simulink model "TB31_R2_ScPause_LoadStop"  (R2025a)
settings: Solver=FixedStepDiscrete  StartTime=0  StopTime=TB.t_end  FixedStep=TB.dt  RelTol=1e-3
InitFcn:
  | % 모델과 같은 폴더의 초기화 스크립트를 실행해 P(설계 파라미터)와 TB(시험 조건)를 만든다.
  | run(fullfile(fileparts(get_param(bdroot, 'FileName')), 'TB31_init.m'));
values from neighbouring files (symbols this model uses):
  TB = struct()    [TB31_init.m]    (also in run_TB31.m = evalin('base', 'TB'))
libraries: fl_lib x71, nesl_utility x31
(part 1 of 3)
settings Model: Creator=hj000  LastModifiedBy=hj000
settings DataIOCC: SaveOutput=off  SignalLogging=off  SaveTime=off

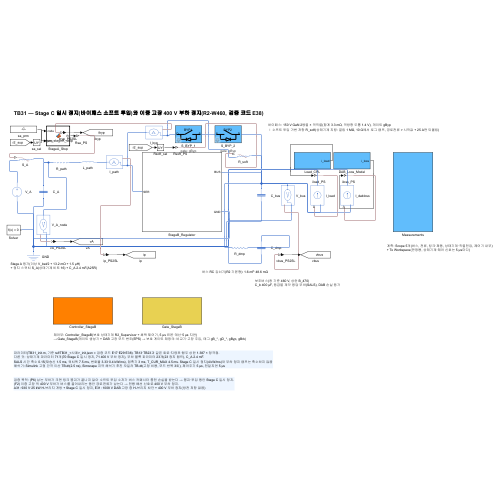
[thumbnail: Simulink's stored preview of the top-level diagram]
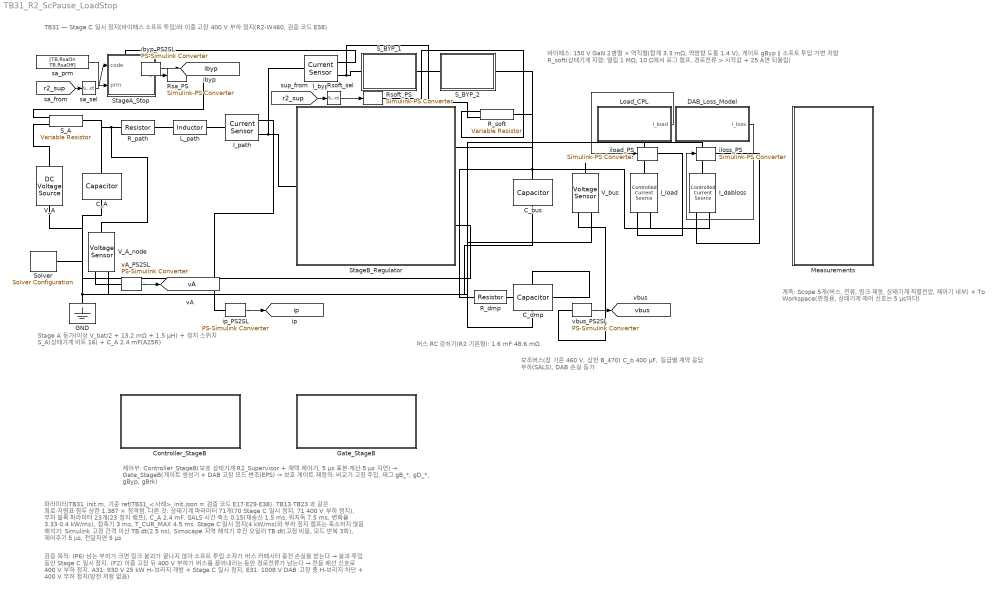
== system TB31_R2_ScPause_LoadStop ==
  note: TB31 — Stage C 일시 정지(바이패스 소프트 투입)와 이중 고장 400 V 부하 정지(R2-W460, 검증 코드 E38)
  note: Stage A 등가(이상 V_bat/2 + 13.2 mΩ + 1.5 µH)
      | + 정지 스위치 S_A(상태기계 비트 16) + C_A 2.4 mF(A25R)
  note: 바이패스: 150 V GaN 2병렬 × 역직렬(합계 3.3 mΩ, 역방향 도통 1.4 V), 게이트 gByp
      | ∥ 소프트 투입 가변 저항 R_soft(상태기계 지령: 열림 1 MΩ, 10 Ω에서 로그 램프, 경로전류 > 시작값 + 25 A면 되올림)
  note: 버스 RC 감쇠기(R2 기본형): 1.6 mF·48.6 mΩ
  note: 보조버스(창 기준 460 V, 상한 B_470)
      | C_b 400 µF, 등급별 계약 응답 부하(SALS), DAB 손실 등가
  note: 제어부: Controller_StageB(보호 상태기계 R2_Supervisor + 채택 제어기, 5 µs 표본·계산·5 µs 지연)
      | → Gate_StageB(게이트 생성기 + DAB 고장 모드 변조(EPS) → 보호 게이트 재정의: 비교기·고장 주입, 태그 gB_*, gD_*, gByp, gBrk)
  note: 계측: Scope 5개(버스, 전류, 링크·제동, 상태기계·직렬전압, 제어기 내부)
      | + To Workspace(판정용, 상태기계·제어 신호는 5 µs마다)
  note: 파라미터(TB31_init.m, 기준 ref/TB31_<사례>_init.json = 검증 코드 E17·E29·E38). TB13·TB23과 같은 회로·지령표·첨두 상한 1.387 × 정격점.
      | 다른 것: 상태기계 파라미터 71개(70 Stage C 일시 정지, 71 400 V 부하 정지), 부하 블록 파라미터 23개(23 정지 램프), C_A 2.4 mF.
      | SALS 시간 축소 0.15(재송신 1.5 ms, 워치독 7.5 ms, 변화율 3.33·0.4 kW/ms), 접촉기 3 ms, T_CUR_MAX 4.5 ms. Stage C 일시 정지(4 kW/ms)와 부하 정지 램프는 축소하지 않음
      | 해석기: Simulink 고정 간격 이산 TB.dt(2.5 ns), Simscape 지역 해석기 후진 오일러 TB.dt(고정 비용, 모드 반복 3회), 제어주기 5 µs, 전달지연 5 µs
  note: 검증 목적: (P6) 남는 부하가 크면 링크 붕괴가 끝나지 않아 소프트 투입 소자가 버스 커패시터 충전 손실을 받는다 → 붕괴·투입 동안 Stage C 일시 정지.
      | (F2) 이중 고장 뒤 400 V 부하가 버스를 끌어내리는 동안 경로전류가 남는다 → 전용 배선 신호로 400 V 부하 정지.
      | A31: 930 V·25 kW H-브리지 개방 + Stage C 일시 정지, E31: 1008 V DAB 고장 중 H-브리지 차단 + 400 V 부하 정지(방전 저항 없음)
  C_A : fl_lib/Electrical/Electrical Elements/Capacitor  c=TB.CA F  r=0 Ohm  g=0 1/Ohm  i_specify=off  i_priority=None  i=0 A  i_nominal_specify=off  i_nominal_value=1  i_nominal_unit=A  v_specify=off  v_priority=None  v=0 V  v_nominal_specify=off  v_nominal_value=1  v_nominal_unit=V  vc_specify=on  vc_priority=High  vc=TB.VA V  vc_nominal_specify=off  vc_nominal_value=1  vc_nominal_unit=V
  C_bus : fl_lib/Electrical/Electrical Elements/Capacitor  c=TB.Cb F  r=1e-6 Ohm  g=0 1/Ohm  i_specify=off  i_priority=None  i=0 A  i_nominal_specify=off  i_nominal_value=1  i_nominal_unit=A  v_specify=off  v_priority=None  v=0 V  v_nominal_specify=off  v_nominal_value=1  v_nominal_unit=V  vc_specify=on  vc_priority=High  vc=TB.vb0 V  vc_nominal_specify=off  vc_nominal_value=1  vc_nominal_unit=V
  C_dmp : fl_lib/Electrical/Electrical Elements/Capacitor  c=TB.Cdmp F  r=0 Ohm  g=0 1/Ohm  i_specify=off  i_priority=None  i=0 A  i_nominal_specify=off  i_nominal_value=1  i_nominal_unit=A  v_specify=off  v_priority=None  v=0 V  v_nominal_specify=off  v_nominal_value=1  v_nominal_unit=V  vc_specify=on  vc_priority=High  vc=TB.vcd0 V  vc_nominal_specify=off  vc_nominal_value=1  vc_nominal_unit=V
  Controller_StageB : Subsystem
  DAB_Loss_Model : Subsystem
  GND : fl_lib/Electrical/Electrical Elements/Electrical Reference
  Gate_StageB : Subsystem
  I_byp : fl_lib/Electrical/Electrical Sensors/Current Sensor
  I_dabloss : fl_lib/Electrical/Electrical Sources/Controlled Current Source
  I_load : fl_lib/Electrical/Electrical Sources/Controlled Current Source
  I_path : fl_lib/Electrical/Electrical Sensors/Current Sensor
  L_path : fl_lib/Electrical/Electrical Elements/Inductor  l=TB.Lpath H  r=0 Ohm  g=1e-9 1/Ohm  i_specify=off  i_priority=None  i=0 A  i_nominal_specify=off  i_nominal_value=1  i_nominal_unit=A  v_specify=off  v_priority=None  v=0 V  v_nominal_specify=off  v_nominal_value=1  v_nominal_unit=V  i_L_specify=on  i_L_priority=High  i_L=TB.ip0 A  i_L_nominal_specify=off  i_L_nominal_value=1  i_L_nominal_unit=A
  Load_CPL : Subsystem
  Measurements : Subsystem
  R_dmp : fl_lib/Electrical/Electrical Elements/Resistor  R=TB.Rdmp Ohm  i_specify=off  i_priority=None  i=0 A  i_nominal_specify=off  i_nominal_value=1  i_nominal_unit=A  v_specify=off  v_priority=None  v=0 V  v_nominal_specify=off  v_nominal_value=1  v_nominal_unit=V
  R_path : fl_lib/Electrical/Electrical Elements/Resistor  R=TB.Rpath Ohm  i_specify=off  i_priority=None  i=0 A  i_nominal_specify=off  i_nominal_value=1  i_nominal_unit=A  v_specify=off  v_priority=None  v=0 V  v_nominal_specify=off  v_nominal_value=1  v_nominal_unit=V
  R_soft : fl_lib/Electrical/Electrical Elements/Variable Resistor  Rmin=1e-4 Ohm  thermalEnable=false  thermal_mass=1 J/K  i_specify=off  i_priority=None  i=0 A  i_nominal_specify=off  i_nominal_value=1  i_nominal_unit=A  v_specify=off  v_priority=None  v=0 V  v_nominal_specify=off  v_nominal_value=1  v_nominal_unit=V  T_specify=off  T_priority=None  T=300 K  T_nominal_specify=off  T_nominal_value=1  T_nominal_unit=K
  Rsa_PS : nesl_utility/Simulink-PS Converter  PhysicalDomain=network_engine_domain  SubClassName=ps_input  LeftPortType=input  RightPortType=output  PseudoPeriodic=off  Frequencies=[]  NoiseDistribution=none  NoiseParameters=[]  Unit=1  AffineConversion=off  FilteringAndDerivatives=provide  SimscapeFilterOrder=1  InputFilterTimeConstant=0.001  UdotUserProvided=0
  Rsoft_PS : nesl_utility/Simulink-PS Converter  PhysicalDomain=network_engine_domain  SubClassName=ps_input  LeftPortType=input  RightPortType=output  PseudoPeriodic=off  Frequencies=[]  NoiseDistribution=none  NoiseParameters=[]  Unit=1  AffineConversion=off  FilteringAndDerivatives=provide  SimscapeFilterOrder=1  InputFilterTimeConstant=0.001  UdotUserProvided=0
  Rsoft_sel : Selector  InputPortWidth=12  IndexOptions=Index vector (dialog)  Indices=7  OutputSizes=1
  S_A : fl_lib/Electrical/Electrical Elements/Variable Resistor  Rmin=1e-5 Ohm  thermalEnable=false  thermal_mass=1 J/K  i_specify=off  i_priority=None  i=0 A  i_nominal_specify=off  i_nominal_value=1  i_nominal_unit=A  v_specify=off  v_priority=None  v=0 V  v_nominal_specify=off  v_nominal_value=1  v_nominal_unit=V  T_specify=off  T_priority=None  T=300 K  T_nominal_specify=off  T_nominal_value=1  T_nominal_unit=K
  S_BYP_1 : Subsystem  mask(PRISM-Hub switch cell){Ron=TB.Rbyp_cell, Goff=TB.B.Goff, Vf=TB.Vf_byp, Rd=TB.Rd_byp, Goffd=TB.B.Goffd}
      mask prompts: Ron "도통 저항 R_on [Ohm]"; Goff "차단 컨덕턴스 G_off [S]"; Vf "다이오드 순방향 전압 Vf [V]"; Rd "다이오드 도통 저항 R_d [Ohm]"; Goffd "다이오드 차단 컨덕턴스 [S]"
      mask help: 전력 반도체 스위치 셀 BYP1. 게이트 태그 gByp.
      settings: AttributesFormatString=gate: gByp
      mask Display:
      | plot([0.05 0.35 ],[0.50 0.50 ],[0.35 0.65 ],[0.50 0.74 ],[0.65 0.95 ],[0.50 0.50 ]);
      | plot([0.20 0.20 0.42 ],[0.50 0.20 0.20 ],[0.58 0.80 0.80 ],[0.20 0.20 0.50 ]);
      | plot([0.42 0.58 0.58 0.42 ],[0.20 0.10 0.30 0.20 ],[0.42 0.42 ],[0.10 0.30 ]);
      | text(0.5,0.80,'BYP1','horizontalAlignment','center','texmode','off');
      | port_label('LConn',1,'D');
      | port_label('RConn',1,'S');
  S_BYP_2 : Subsystem  mask(PRISM-Hub switch cell){Ron=TB.Rbyp_cell, Goff=TB.B.Goff, Vf=TB.Vf_byp, Rd=TB.Rd_byp, Goffd=TB.B.Goffd}
      mask prompts: Ron "도통 저항 R_on [Ohm]"; Goff "차단 컨덕턴스 G_off [S]"; Vf "다이오드 순방향 전압 Vf [V]"; Rd "다이오드 도통 저항 R_d [Ohm]"; Goffd "다이오드 차단 컨덕턴스 [S]"
      mask help: 전력 반도체 스위치 셀 BYP2. 게이트 태그 gByp.
      settings: AttributesFormatString=gate: gByp
      mask Display:
      | plot([0.95 0.65 ],[0.50 0.50 ],[0.65 0.35 ],[0.50 0.74 ],[0.35 0.05 ],[0.50 0.50 ]);
      | plot([0.80 0.80 0.58 ],[0.50 0.20 0.20 ],[0.42 0.20 0.20 ],[0.20 0.20 0.50 ]);
      | plot([0.58 0.42 0.42 0.58 ],[0.20 0.10 0.30 0.20 ],[0.58 0.58 ],[0.10 0.30 ]);
      | text(0.5,0.80,'BYP2','horizontalAlignment','center','texmode','off');
      | port_label('LConn',1,'D');
      | port_label('RConn',1,'S');
  Solver : nesl_utility/Solver Configuration  PhysicalDomain=network_engine_domain  SubClassName=solver  LeftPortType=input  RightPortType=generic  Tones=[]  Harmonics=[]  SimulateNoise=off  Profile=off  UseLocalSampling=off  EnableSwitchedLinearOptims=on  FrequencyDomain=off  UseCCode=off  RelTol=0.001  AbsTol=0.001  MinStep=1e-09  ToWorkspace=off  RevertToSquareIcSolve=off  NumHomotopyIterations=100  PhasorMode=off  PhasorModeNumHarmonics=1  ConsistencySolver=NEWTON_XTOL_AFTER_FTOL  IndexReductionMethod=DerivativeReplacement  DoDC=off  ResidualTolerance=1e-9  ConsistencyTolSource=GLOBAL  ConsistencyAbsTol=0.001  ConsistencyRelTol=0.001  ConsistencyTolFactor=0.001  UseLocalSolver=on  LocalSolverChoice=NE_BACKWARD_EULER_ADVANCER  ResolveIndetEquations=on  FunctionEvalNumThread=1  LocalSolverSampleTime=TB.dt  DoFixedCost=on  MaxNonlinIter=3  MaxModeIter=2  ComputeImpulses=off  ImpulseIterations=2  LinearAlgebra=auto  LinearAlgebraNumThread=0  EquationFormulation=NE_TIME_EF  DelaysMemoryBudget=1024  AutomaticFiltering=on  FilteringTimeConstant=0.001  PartitionStorageMethod=AS_NEEDED  PartitionMemoryBudget=1024  PartitionMethod=ROBUST  MultibodyUseLocalSolver=off  MultibodyLocalSolverChoice=ODE1  MultibodyLocalSolverSampleTime=0.001
  StageA_Stop : MATLAB Function  TreatAsAtomicUnit=on
  StageB_Regulator : Subsystem
  V_A : fl_lib/Electrical/Electrical Sources/DC Voltage Source  v0=TB.VA V
  V_A_node : fl_lib/Electrical/Electrical Sensors/Voltage Sensor
  V_bus : fl_lib/Electrical/Electrical Sensors/Voltage Sensor
  ibyp_PS2SL : nesl_utility/PS-Simulink Converter  PhysicalDomain=network_engine_domain  SubClassName=ps_output  LeftPortType=input  RightPortType=output  PseudoPeriodic=off  Frequencies=[]  VectorFormat=inherit  Unit=inherit  AffineConversion=off
  iload_PS : nesl_utility/Simulink-PS Converter  PhysicalDomain=network_engine_domain  SubClassName=ps_input  LeftPortType=input  RightPortType=output  PseudoPeriodic=off  Frequencies=[]  NoiseDistribution=none  NoiseParameters=[]  Unit=1  AffineConversion=off  FilteringAndDerivatives=provide  SimscapeFilterOrder=1  InputFilterTimeConstant=0.001  UdotUserProvided=0
  iloss_PS : nesl_utility/Simulink-PS Converter  PhysicalDomain=network_engine_domain  SubClassName=ps_input  LeftPortType=input  RightPortType=output  PseudoPeriodic=off  Frequencies=[]  NoiseDistribution=none  NoiseParameters=[]  Unit=1  AffineConversion=off  FilteringAndDerivatives=provide  SimscapeFilterOrder=1  InputFilterTimeConstant=0.001  UdotUserProvided=0
  ip_PS2SL : nesl_utility/PS-Simulink Converter  PhysicalDomain=network_engine_domain  SubClassName=ps_output  LeftPortType=input  RightPortType=output  PseudoPeriodic=off  Frequencies=[]  VectorFormat=inherit  Unit=inherit  AffineConversion=off
  sa_prm : Constant  Value=[TB.RsaOn TB.RsaOff]
  sa_sel : Selector  InputPortWidth=12  IndexOptions=Index vector (dialog)  Indices=10  OutputSizes=1
  vA_PS2SL : nesl_utility/PS-Simulink Converter  PhysicalDomain=network_engine_domain  SubClassName=ps_output  LeftPortType=input  RightPortType=output  PseudoPeriodic=off  Frequencies=[]  VectorFormat=inherit  Unit=inherit  AffineConversion=off
  vbus_PS2SL : nesl_utility/PS-Simulink Converter  PhysicalDomain=network_engine_domain  SubClassName=ps_output  LeftPortType=input  RightPortType=output  PseudoPeriodic=off  Frequencies=[]  VectorFormat=inherit  Unit=inherit  AffineConversion=off
  tag scope: ibyp=global, ip=global, vA=global, vbus=global
  wires:
  [r2_sup] -> sa_sel/1
  sa_sel/1 -> StageA_Stop/1(code)
  sa_prm/1 -> StageA_Stop/2(prm)
  StageA_Stop/1(R) -> Rsa_PS/1
  [r2_sup] -> Rsoft_sel/1
  Rsoft_sel/1 -> Rsoft_PS/1
  ip_PS2SL/1 -> [ip]
  vbus_PS2SL/1 -> [vbus]
  ibyp_PS2SL/1 -> [ibyp]
  vA_PS2SL/1 -> [vA]
  Load_CPL/1(i_load) -> iload_PS/1
  DAB_Loss_Model/1(i_loss) -> iloss_PS/1
  connections:
  Solver/RConn1 -- C_A/RConn1 -- V_A_node/RConn2 -- V_A/RConn1 -- StageB_Regulator/RConn2 -- C_bus/RConn1 -- C_dmp/RConn1 -- V_bus/RConn2 -- I_load/LConn1 -- GND/LConn1 -- I_dabloss/LConn1
  V_A/LConn1 -- S_A/LConn2
  S_A/RConn1 -- C_A/LConn1 -- R_path/LConn1 -- V_A_node/LConn1
  Rsa_PS/RConn1 -- S_A/LConn1
  R_path/RConn1 -- L_path/LConn1
  L_path/RConn1 -- I_path/LConn1
  StageB_Regulator/LConn1 -- I_path/RConn2 -- I_byp/LConn1
  S_BYP_1/LConn1 -- I_byp/RConn2 -- R_soft/LConn2
  S_BYP_1/RConn1 -- S_BYP_2/RConn1
  S_BYP_2/LConn1 -- R_soft/RConn1 -- StageB_Regulator/RConn1 -- R_dmp/LConn1 -- V_bus/LConn1 -- I_load/RConn2 -- C_bus/LConn1 -- I_dabloss/RConn2
  Rsoft_PS/RConn1 -- R_soft/LConn1
  R_dmp/RConn1 -- C_dmp/LConn1
  iload_PS/RConn1 -- I_load/RConn1
  iloss_PS/RConn1 -- I_dabloss/RConn1
  I_path/RConn1 -- ip_PS2SL/LConn1
  V_bus/RConn1 -- vbus_PS2SL/LConn1
  I_byp/RConn1 -- ibyp_PS2SL/LConn1
  V_A_node/RConn1 -- vA_PS2SL/LConn1

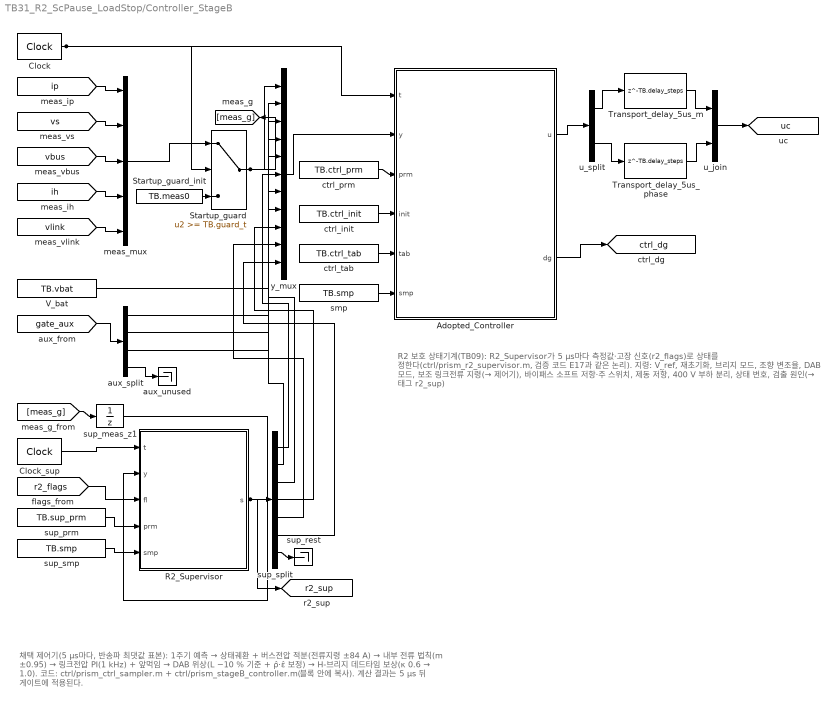
== system TB31_R2_ScPause_LoadStop/Controller_StageB ==
  note: R2 보호 상태기계(TB09): R2_Supervisor가 5 µs마다 측정값·고장 신호(r2_flags)로 상태를 정한다(ctrl/prism_r2_supervisor.m,
      | 검증 코드 E17과 같은 논리). 지령: V_ref, 재초기화, 브리지 모드, 조향 변조율, DAB 모드, 보조 링크전류 지령(→ 제어기),
      | 바이패스 소프트 저항·주 스위치, 제동 저항, 400 V 부하 분리, 상태 번호, 검출 원인(→ 태그 r2_sup)
  note: 채택 제어기(5 µs마다, 반송파 최댓값 표본): 1주기 예측 → 상태궤환 + 버스전압 적분(전류지령 ±84 A) → 내부 전류 법칙(m ±0.95)
      | → 링크전압 PI(1 kHz) + 앞먹임 → DAB 위상(L −10 % 기준 + ρ̂·ε̂ 보정) → H-브리지 데드타임 보상(κ 0.6 → 1.0).
      | 코드: ctrl/prism_ctrl_sampler.m + ctrl/prism_stageB_controller.m(블록 안에 복사). 계산 결과는 5 µs 뒤 게이트에 적용된다.
  Adopted_Controller : MATLAB Function  TreatAsAtomicUnit=on
  Clock : DigitalClock  SampleTime=TB.dt
  Clock_sup : DigitalClock  SampleTime=TB.dt
  R2_Supervisor : MATLAB Function  TreatAsAtomicUnit=on
  Startup_guard : Switch  Threshold=TB.guard_t  SaturateOnIntegerOverflow=off  InputSameDT=off
  Startup_guard_init : Constant  Value=TB.meas0
  Transport_delay_5us_m : Delay  DelayLength=TB.delay_steps  InitialCondition=TB.uc0(1)
  Transport_delay_5us_phase : Delay  DelayLength=TB.delay_steps  InitialCondition=TB.uc0(2)
  V_bat : Constant  Value=TB.vbat
  aux_split : Demux  Outputs=[1 1 1 3]
  aux_unused : Terminator
  ctrl_init : Constant  Value=TB.ctrl_init
  ctrl_prm : Constant  Value=TB.ctrl_prm
  ctrl_tab : Constant  Value=TB.ctrl_tab
  meas_mux : Mux  Inputs=5
  smp : Constant  Value=TB.smp
  sup_meas_z1 : UnitDelay  InitialCondition=TB.meas0'  SampleTime=TB.dt  HasFrameUpgradeWarning=on
  sup_prm : Constant  Value=TB.sup_prm
  sup_rest : Terminator
  sup_smp : Constant  Value=TB.smp
  sup_split : Demux  Outputs=[1 1 1 1 1 1 6]
  u_join : Mux  Inputs=2
  u_split : Demux  Outputs=2
  y_mux : Mux  Inputs=11
  tag scope: ctrl_dg=global, r2_sup=global, uc=global
  wires:
  [ip] -> meas_mux/1
  [vs] -> meas_mux/2
  [vbus] -> meas_mux/3
  [ih] -> meas_mux/4
  [vlink] -> meas_mux/5
  Startup_guard_init/1 -> Startup_guard/3
  meas_mux/1 -> Startup_guard/1
  Clock/1 -> Startup_guard/2, Adopted_Controller/1(t)
  Startup_guard/1 -> y_mux/1, [meas_g]
  V_bat/1 -> y_mux/2
  [gate_aux] -> aux_split/1
  aux_split/1 -> y_mux/3
  aux_split/2 -> y_mux/4
  aux_split/3 -> y_mux/5
  aux_split/4 -> aux_unused/1
  Clock_sup/1 -> R2_Supervisor/1(t)
  [meas_g] -> sup_meas_z1/1
  sup_meas_z1/1 -> R2_Supervisor/2(y)
  [r2_flags] -> R2_Supervisor/3(fl)
  sup_prm/1 -> R2_Supervisor/4(prm)
  sup_smp/1 -> R2_Supervisor/5(smp)
  R2_Supervisor/1(s) -> [r2_sup], sup_split/1
  sup_split/1 -> y_mux/6
  sup_split/2 -> y_mux/7
  sup_split/3 -> y_mux/8
  sup_split/4 -> y_mux/9
  sup_split/5 -> y_mux/10
  sup_split/6 -> y_mux/11
  sup_split/7 -> sup_rest/1
  y_mux/1 -> Adopted_Controller/2(y)
  ctrl_prm/1 -> Adopted_Controller/3(prm)
  ctrl_init/1 -> Adopted_Controller/4(init)
  ctrl_tab/1 -> Adopted_Controller/5(tab)
  smp/1 -> Adopted_Controller/6(smp)
  Adopted_Controller/1(u) -> u_split/1
  u_split/1 -> Transport_delay_5us_m/1
  u_split/2 -> Transport_delay_5us_phase/1
  Transport_delay_5us_m/1 -> u_join/1
  Transport_delay_5us_phase/1 -> u_join/2
  u_join/1 -> [uc]
  Adopted_Controller/2(dg) -> [ctrl_dg]

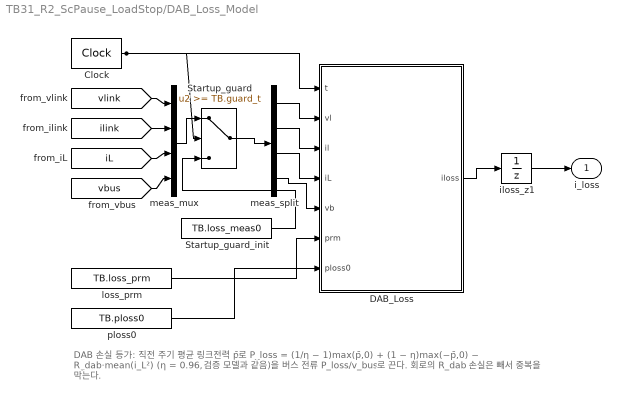
== system TB31_R2_ScPause_LoadStop/DAB_Loss_Model ==
  note: DAB 손실 등가: 직전 주기 평균 링크전력 p̄로 P_loss = (1/η − 1)max(p̄,0) + (1 − η)max(−p̄,0) − R_dab·mean(i_L²)
      | (η = 0.96, 검증 모델과 같음)을 버스 전류 P_loss/v_bus로 끈다. 회로의 R_dab 손실은 빼서 중복을 막는다.
  Clock : DigitalClock  SampleTime=TB.dt
  DAB_Loss : MATLAB Function  TreatAsAtomicUnit=on
  Startup_guard : Switch  Threshold=TB.guard_t  SaturateOnIntegerOverflow=off  InputSameDT=off
  Startup_guard_init : Constant  Value=TB.loss_meas0
  iloss_z1 : UnitDelay  SampleTime=TB.dt  HasFrameUpgradeWarning=on
  loss_prm : Constant  Value=TB.loss_prm
  meas_mux : Mux
  meas_split : Demux
  ploss0 : Constant  Value=TB.ploss0
  i_loss : Outport
  wires:
  [vlink] -> meas_mux/1
  [ilink] -> meas_mux/2
  [iL] -> meas_mux/3
  [vbus] -> meas_mux/4
  Startup_guard_init/1 -> Startup_guard/3
  meas_mux/1 -> Startup_guard/1
  Clock/1 -> Startup_guard/2, DAB_Loss/1(t)
  Startup_guard/1 -> meas_split/1
  meas_split/1 -> DAB_Loss/2(vl)
  meas_split/2 -> DAB_Loss/3(il)
  meas_split/3 -> DAB_Loss/4(iL)
  meas_split/4 -> DAB_Loss/5(vb)
  loss_prm/1 -> DAB_Loss/6(prm)
  ploss0/1 -> DAB_Loss/7(ploss0)
  DAB_Loss/1(iloss) -> iloss_z1/1
  iloss_z1/1 -> i_loss/1

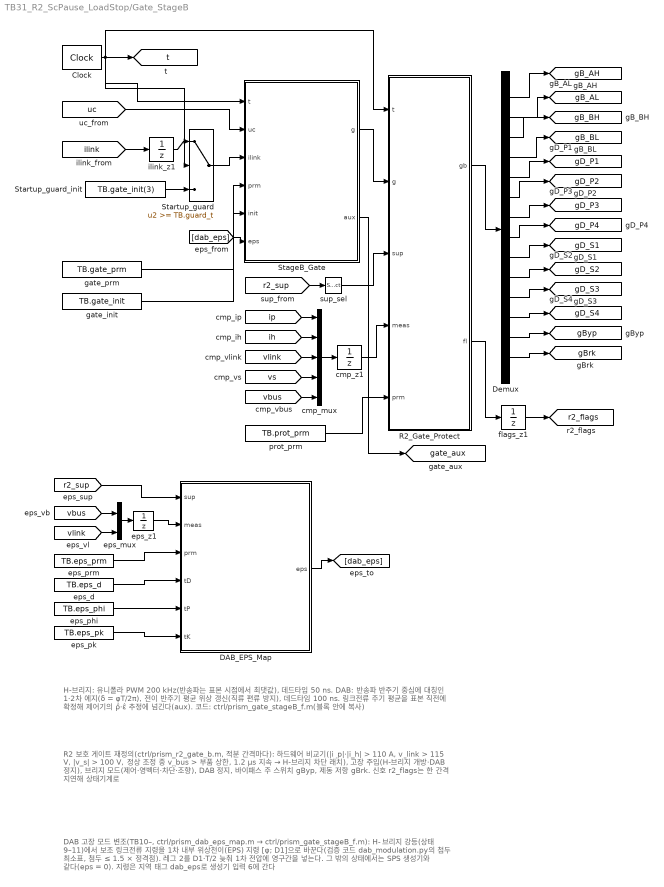
== system TB31_R2_ScPause_LoadStop/Gate_StageB ==
  note: H-브리지: 유니폴라 PWM 200 kHz(반송파는 표본 시점에서 최댓값), 데드타임 50 ns.
      | DAB: 반송파 반주기 중심에 대칭인 1·2차 에지(δ = φT/2π), 전이 반주기 평균 위상 갱신(직류 편류 방지), 데드타임 100 ns.
      | 링크전류 주기 평균을 표본 직전에 확정해 제어기의 ρ̂·ε̂ 추정에 넘긴다(aux). 코드: ctrl/prism_gate_stageB_f.m(블록 안에 복사)
  note: DAB 고장 모드 변조(TB10–, ctrl/prism_dab_eps_map.m → ctrl/prism_gate_stageB_f.m): H-브리지 강등(상태 9–11)에서 보조 링크전류 지령을
      | 1차 내부 위상천이(EPS) 지령 [φ; D1]으로 바꾼다(검증 코드 dab_modulation.py의 첨두 최소표, 첨두 ≤ 1.5 × 정격점). 레그 2를 D1·T/2 늦춰
      | 1차 전압에 영구간을 넣는다. 그 밖의 상태에서는 SPS 생성기와 같다(eps = 0). 지령은 지역 태그 dab_eps로 생성기 입력 6에 간다
  note: R2 보호 게이트 재정의(ctrl/prism_r2_gate_b.m, 적분 간격마다): 하드웨어 비교기(|i_p|·|i_h| > 110 A, v_link > 115 V,
      | |v_s| > 100 V, 정상 조정 중 v_bus > 부품 상한, 1.2 µs 지속 → H-브리지 차단 래치), 고장 주입(H-브리지 개방·DAB 정지),
      | 브리지 모드(제어·영벡터·차단·조향), DAB 정지, 바이패스 주 스위치 gByp, 제동 저항 gBrk. 신호 r2_flags는 한 간격 지연해 상태기계로
  Clock : DigitalClock  SampleTime=TB.dt
  DAB_EPS_Map : MATLAB Function  TreatAsAtomicUnit=on
  Demux : Demux  Outputs=14
  R2_Gate_Protect : MATLAB Function  TreatAsAtomicUnit=on
  StageB_Gate : MATLAB Function  TreatAsAtomicUnit=on
  Startup_guard : Switch  Threshold=TB.guard_t  SaturateOnIntegerOverflow=off  InputSameDT=off
  Startup_guard_init : Constant  Value=TB.gate_init(3)
  cmp_mux : Mux  Inputs=5
  cmp_z1 : UnitDelay  InitialCondition=[TB.ip0 TB.ih0 TB.vl0 TB.vs0 TB.vb0]'  SampleTime=TB.dt  HasFrameUpgradeWarning=on
  eps_d : Constant  Value=TB.eps_d
  eps_mux : Mux  Inputs=2
  eps_phi : Constant  Value=TB.eps_phi
  eps_pk : Constant  Value=TB.eps_pk
  eps_prm : Constant  Value=TB.eps_prm
  eps_z1 : UnitDelay  InitialCondition=[TB.vb0 TB.vl0]'  SampleTime=TB.dt  HasFrameUpgradeWarning=on
  flags_z1 : UnitDelay  SampleTime=TB.dt  HasFrameUpgradeWarning=on
  gate_init : Constant  Value=TB.gate_init
  gate_prm : Constant  Value=TB.gate_prm
  ilink_z1 : UnitDelay  SampleTime=TB.dt  HasFrameUpgradeWarning=on
  prot_prm : Constant  Value=TB.prot_prm
  sup_sel : Selector  InputPortWidth=12  IndexOptions=Index vector (dialog)  Indices=[3 5 8 9 11]  OutputSizes=1
  tag scope: gB_AH=global, gB_AL=global, gB_BH=global, gB_BL=global, gBrk=global, gByp=global, gD_P1=global, gD_P2=global, gD_P3=global, gD_P4=global, gD_S1=global, gD_S2=global, gD_S3=global, gD_S4=global, gate_aux=global, r2_flags=global, t=global
  wires:
  Startup_guard_init/1 -> Startup_guard/3
  Clock/1 -> [t], StageB_Gate/1(t), Startup_guard/2, R2_Gate_Protect/1(t)
  [uc] -> StageB_Gate/2(uc)
  [ilink] -> ilink_z1/1
  ilink_z1/1 -> Startup_guard/1
  Startup_guard/1 -> StageB_Gate/3(ilink)
  gate_prm/1 -> StageB_Gate/4(prm)
  gate_init/1 -> StageB_Gate/5(init)
  [r2_sup] -> sup_sel/1
  [ip] -> cmp_mux/1
  [ih] -> cmp_mux/2
  [vlink] -> cmp_mux/3
  [vs] -> cmp_mux/4
  [vbus] -> cmp_mux/5
  cmp_mux/1 -> cmp_z1/1
  StageB_Gate/1(g) -> R2_Gate_Protect/2(g)
  sup_sel/1 -> R2_Gate_Protect/3(sup)
  cmp_z1/1 -> R2_Gate_Protect/4(meas)
  prot_prm/1 -> R2_Gate_Protect/5(prm)
  R2_Gate_Protect/1(gb) -> Demux/1
  R2_Gate_Protect/2(fl) -> flags_z1/1
  flags_z1/1 -> [r2_flags]
  [vbus] -> eps_mux/1
  [vlink] -> eps_mux/2
  eps_mux/1 -> eps_z1/1
  [r2_sup] -> DAB_EPS_Map/1(sup)
  eps_z1/1 -> DAB_EPS_Map/2(meas)
  eps_prm/1 -> DAB_EPS_Map/3(prm)
  eps_d/1 -> DAB_EPS_Map/4(tD)
  eps_phi/1 -> DAB_EPS_Map/5(tP)
  eps_pk/1 -> DAB_EPS_Map/6(tK)
  DAB_EPS_Map/1(eps) -> [dab_eps]
  [dab_eps] -> StageB_Gate/6(eps)
  Demux/1 -> [gB_AH]
  Demux/2 -> [gB_AL]
  Demux/3 -> [gB_BH]
  Demux/4 -> [gB_BL]
  Demux/5 -> [gD_P1]
  Demux/6 -> [gD_P2]
  Demux/7 -> [gD_P3]
  Demux/8 -> [gD_P4]
  Demux/9 -> [gD_S1]
  Demux/10 -> [gD_S2]
  Demux/11 -> [gD_S3]
  Demux/12 -> [gD_S4]
  Demux/13 -> [gByp]
  Demux/14 -> [gBrk]
  StageB_Gate/2(aux) -> [gate_aux]

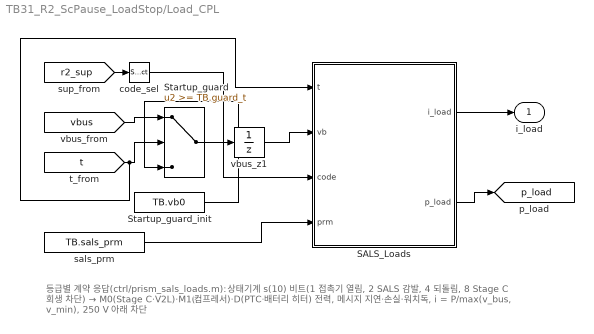
== system TB31_R2_ScPause_LoadStop/Load_CPL ==
  note: 등급별 계약 응답(ctrl/prism_sals_loads.m): 상태기계 s(10) 비트(1 접촉기 열림, 2 SALS 감발, 4 되돌림, 8 Stage C 회생 차단)
      | → M0(Stage C·V2L)·M1(컴프레서)·D(PTC·배터리 히터) 전력, 메시지 지연·손실·워치독, i = P/max(v_bus, v_min), 250 V 아래 차단
  SALS_Loads : MATLAB Function  TreatAsAtomicUnit=on
  Startup_guard : Switch  Threshold=TB.guard_t  SaturateOnIntegerOverflow=off  InputSameDT=off
  Startup_guard_init : Constant  Value=TB.vb0
  code_sel : Selector  InputPortWidth=12  IndexOptions=Index vector (dialog)  Indices=10  OutputSizes=1
  sals_prm : Constant  Value=TB.sals_prm
  vbus_z1 : UnitDelay  SampleTime=TB.dt  HasFrameUpgradeWarning=on
  i_load : Outport
  tag scope: p_load=global
  wires:
  [r2_sup] -> code_sel/1
  Startup_guard_init/1 -> Startup_guard/3
  [vbus] -> Startup_guard/1
  [t] -> Startup_guard/2, SALS_Loads/1(t)
  Startup_guard/1 -> vbus_z1/1
  vbus_z1/1 -> SALS_Loads/2(vb)
  code_sel/1 -> SALS_Loads/3(code)
  sals_prm/1 -> SALS_Loads/4(prm)
  SALS_Loads/1(i_load) -> i_load/1
  SALS_Loads/2(p_load) -> [p_load]

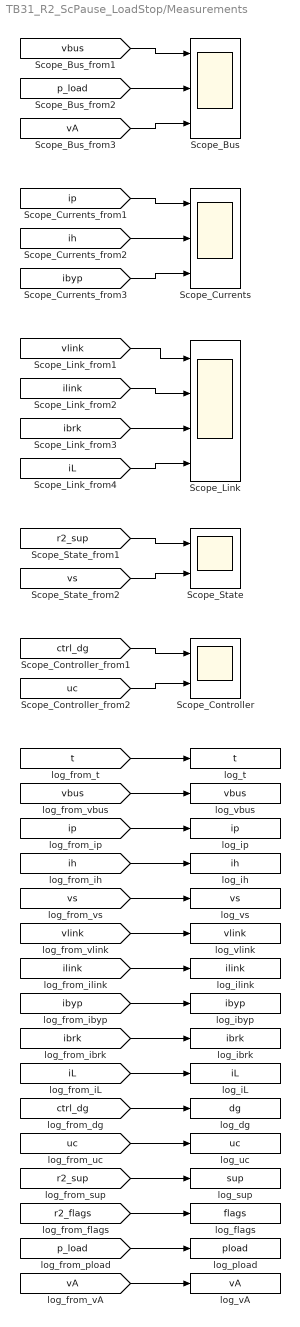
== system TB31_R2_ScPause_LoadStop/Measurements ==
  Scope_Bus : Scope  NumInputPorts=3
      settings: Title=Scope Bus
  Scope_Controller : Scope  NumInputPorts=2
      settings: Title=Scope Controller
  Scope_Currents : Scope  NumInputPorts=3
      settings: Title=Scope Currents
  Scope_Link : Scope  NumInputPorts=4
      settings: Title=Scope Link
  Scope_State : Scope  NumInputPorts=2
      settings: Title=Scope State
  log_dg : ToWorkspace  VariableName=dg  SampleTime=-1
      settings: Decimation=TB.Np
  log_flags : ToWorkspace  VariableName=flags  SampleTime=-1
      settings: Decimation=TB.Np
  log_iL : ToWorkspace  VariableName=iL  SampleTime=-1
  log_ibrk : ToWorkspace  VariableName=ibrk  SampleTime=-1
  log_ibyp : ToWorkspace  VariableName=ibyp  SampleTime=-1
  log_ih : ToWorkspace  VariableName=ih  SampleTime=-1
  log_ilink : ToWorkspace  VariableName=ilink  SampleTime=-1
  log_ip : ToWorkspace  VariableName=ip  SampleTime=-1
  log_pload : ToWorkspace  VariableName=pload  SampleTime=-1
      settings: Decimation=TB.Np
  log_sup : ToWorkspace  VariableName=sup  SampleTime=-1
      settings: Decimation=TB.Np
  log_t : ToWorkspace  VariableName=t  SampleTime=-1
  log_uc : ToWorkspace  VariableName=uc  SampleTime=-1
      settings: Decimation=TB.Np
  log_vA : ToWorkspace  VariableName=vA  SampleTime=-1
      settings: Decimation=TB.Np
  log_vbus : ToWorkspace  VariableName=vbus  SampleTime=-1
  log_vlink : ToWorkspace  VariableName=vlink  SampleTime=-1
  log_vs : ToWorkspace  VariableName=vs  SampleTime=-1
  wires:
  [vbus] -> Scope_Bus/1
  [p_load] -> Scope_Bus/2
  [vA] -> Scope_Bus/3
  [ip] -> Scope_Currents/1
  [ih] -> Scope_Currents/2
  [ibyp] -> Scope_Currents/3
  [vlink] -> Scope_Link/1
  [ilink] -> Scope_Link/2
  [ibrk] -> Scope_Link/3
  [iL] -> Scope_Link/4
  [r2_sup] -> Scope_State/1
  [vs] -> Scope_State/2
  [ctrl_dg] -> Scope_Controller/1
  [uc] -> Scope_Controller/2
  [t] -> log_t/1
  [vbus] -> log_vbus/1
  [ip] -> log_ip/1
  [ih] -> log_ih/1
  [vs] -> log_vs/1
  [vlink] -> log_vlink/1
  [ilink] -> log_ilink/1
  [ibyp] -> log_ibyp/1
  [ibrk] -> log_ibrk/1
  [iL] -> log_iL/1
  [ctrl_dg] -> log_dg/1
  [uc] -> log_uc/1
  [r2_sup] -> log_sup/1
  [r2_flags] -> log_flags/1
  [p_load] -> log_pload/1
  [vA] -> log_vA/1

== system TB31_R2_ScPause_LoadStop/S_BYP_1 ==
  note: 스위치 셀: 이상 스위치(R_on, G_off) + 역병렬 바디 다이오드(Vf, R_d)
      | 게이트: 전역 태그 "gByp" (> 0.5 이면 도통)
  D_body : fl_lib/Electrical/Electrical Elements/Diode  Vf=Vf V  Ron=Rd Ohm  Goff=Goffd 1/Ohm  i_specify=off  i_priority=None  i=0 A  i_nominal_specify=off  i_nominal_value=1  i_nominal_unit=A  v_specify=off  v_priority=None  v=0 V  v_nominal_specify=off  v_nominal_value=1  v_nominal_unit=V
  Gate_PS : nesl_utility/Simulink-PS Converter  PhysicalDomain=network_engine_domain  SubClassName=ps_input  LeftPortType=input  RightPortType=output  PseudoPeriodic=off  Frequencies=[]  NoiseDistribution=none  NoiseParameters=[]  Unit=1  AffineConversion=off  FilteringAndDerivatives=zero  SimscapeFilterOrder=1  InputFilterTimeConstant=0.001  UdotUserProvided=0
  SW : fl_lib/Electrical/Electrical Elements/Switch  R_closed=Ron Ohm  G_open=Goff 1/Ohm  Threshold=0.5  i_specify=off  i_priority=None  i=0 A  i_nominal_specify=off  i_nominal_value=1  i_nominal_unit=A  v_specify=off  v_priority=None  v=0 V  v_nominal_specify=off  v_nominal_value=1  v_nominal_unit=V
  D : PMIOPort  Side=Left
  S : PMIOPort  Port=2  Side=Right
  wires:
  [gByp] -> Gate_PS/1
  connections:
  Gate_PS/RConn1 -- SW/RConn1
  SW/LConn1 -- D/RConn1 -- D_body/RConn1
  S/RConn1 -- SW/RConn2 -- D_body/LConn1

== system TB31_R2_ScPause_LoadStop/S_BYP_2 ==
  note: 스위치 셀: 이상 스위치(R_on, G_off) + 역병렬 바디 다이오드(Vf, R_d)
      | 게이트: 전역 태그 "gByp" (> 0.5 이면 도통)
  D_body : fl_lib/Electrical/Electrical Elements/Diode  Vf=Vf V  Ron=Rd Ohm  Goff=Goffd 1/Ohm  i_specify=off  i_priority=None  i=0 A  i_nominal_specify=off  i_nominal_value=1  i_nominal_unit=A  v_specify=off  v_priority=None  v=0 V  v_nominal_specify=off  v_nominal_value=1  v_nominal_unit=V
  Gate_PS : nesl_utility/Simulink-PS Converter  PhysicalDomain=network_engine_domain  SubClassName=ps_input  LeftPortType=input  RightPortType=output  PseudoPeriodic=off  Frequencies=[]  NoiseDistribution=none  NoiseParameters=[]  Unit=1  AffineConversion=off  FilteringAndDerivatives=zero  SimscapeFilterOrder=1  InputFilterTimeConstant=0.001  UdotUserProvided=0
  SW : fl_lib/Electrical/Electrical Elements/Switch  R_closed=Ron Ohm  G_open=Goff 1/Ohm  Threshold=0.5  i_specify=off  i_priority=None  i=0 A  i_nominal_specify=off  i_nominal_value=1  i_nominal_unit=A  v_specify=off  v_priority=None  v=0 V  v_nominal_specify=off  v_nominal_value=1  v_nominal_unit=V
  D : PMIOPort  Side=Left
  S : PMIOPort  Port=2  Side=Right
  wires:
  [gByp] -> Gate_PS/1
  connections:
  Gate_PS/RConn1 -- SW/RConn1
  SW/LConn1 -- D/RConn1 -- D_body/RConn1
  S/RConn1 -- SW/RConn2 -- D_body/LConn1

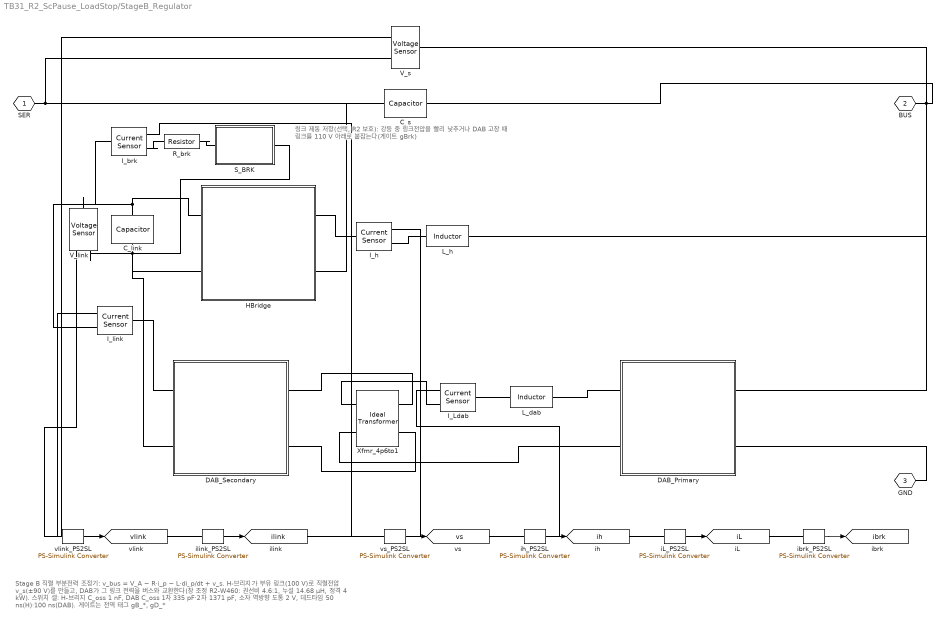
== system TB31_R2_ScPause_LoadStop/StageB_Regulator ==
  note: 링크 제동 저항(선택, R2 보호): 강등 중 링크전압을 빨리 낮추거나
      | DAB 고장 때 링크를 110 V 아래로 붙잡는다(게이트 gBrk)
  note: Stage B 직렬 부분전력 조정기: v_bus = V_A − R·i_p − L·di_p/dt + v_s.
      | H-브리지가 부유 링크(100 V)로 직렬전압 v_s(±90 V)를 만들고, DAB가 그 링크 전력을 버스와 교환한다(창 조정 R2-W460: 권선비 4.6:1, 누설 14.68 µH, 정격 4 kW).
      | 스위치 셀: H-브리지 C_oss 1 nF, DAB C_oss 1차 335 pF·2차 1371 pF, 소자 역방향 도통 2 V, 데드타임 50 ns(H)·100 ns(DAB). 게이트는 전역 태그 gB_*, gD_*
  C_link : fl_lib/Electrical/Electrical Elements/Capacitor  c=TB.B.Clink F  r=1e-6 Ohm  g=0 1/Ohm  i_specify=off  i_priority=None  i=0 A  i_nominal_specify=off  i_nominal_value=1  i_nominal_unit=A  v_specify=off  v_priority=None  v=0 V  v_nominal_specify=off  v_nominal_value=1  v_nominal_unit=V  vc_specify=on  vc_priority=High  vc=TB.vl0 V  vc_nominal_specify=off  vc_nominal_value=1  vc_nominal_unit=V
  C_s : fl_lib/Electrical/Electrical Elements/Capacitor  c=TB.B.Cs F  r=1e-6 Ohm  g=0 1/Ohm  i_specify=off  i_priority=None  i=0 A  i_nominal_specify=off  i_nominal_value=1  i_nominal_unit=A  v_specify=off  v_priority=None  v=0 V  v_nominal_specify=off  v_nominal_value=1  v_nominal_unit=V  vc_specify=on  vc_priority=High  vc=TB.vs0 V  vc_nominal_specify=off  vc_nominal_value=1  vc_nominal_unit=V
  DAB_Primary : Subsystem
  DAB_Secondary : Subsystem
  HBridge : Subsystem
  I_Ldab : fl_lib/Electrical/Electrical Sensors/Current Sensor
  I_brk : fl_lib/Electrical/Electrical Sensors/Current Sensor
  I_h : fl_lib/Electrical/Electrical Sensors/Current Sensor
  I_link : fl_lib/Electrical/Electrical Sensors/Current Sensor
  L_dab : fl_lib/Electrical/Electrical Elements/Inductor  l=TB.B.Ldab H  r=TB.B.Rdab Ohm  g=1e-9 1/Ohm  i_specify=off  i_priority=None  i=0 A  i_nominal_specify=off  i_nominal_value=1  i_nominal_unit=A  v_specify=off  v_priority=None  v=0 V  v_nominal_specify=off  v_nominal_value=1  v_nominal_unit=V  i_L_specify=on  i_L_priority=High  i_L=0 A  i_L_nominal_specify=off  i_L_nominal_value=1  i_L_nominal_unit=A
  L_h : fl_lib/Electrical/Electrical Elements/Inductor  l=TB.B.Lh H  r=TB.B.Rh Ohm  g=1e-9 1/Ohm  i_specify=off  i_priority=None  i=0 A  i_nominal_specify=off  i_nominal_value=1  i_nominal_unit=A  v_specify=off  v_priority=None  v=0 V  v_nominal_specify=off  v_nominal_value=1  v_nominal_unit=V  i_L_specify=on  i_L_priority=High  i_L=TB.ih0 A  i_L_nominal_specify=off  i_L_nominal_value=1  i_L_nominal_unit=A
  R_brk : fl_lib/Electrical/Electrical Elements/Resistor  R=TB.Rbrk Ohm  i_specify=off  i_priority=None  i=0 A  i_nominal_specify=off  i_nominal_value=1  i_nominal_unit=A  v_specify=off  v_priority=None  v=0 V  v_nominal_specify=off  v_nominal_value=1  v_nominal_unit=V
  S_BRK : Subsystem  mask(PRISM-Hub switch cell){Ron=TB.B.Ron, Goff=TB.B.Goff, Vf=TB.B.Vf, Rd=TB.B.Rd, Goffd=TB.B.Goffd}
      mask prompts: Ron "도통 저항 R_on [Ohm]"; Goff "차단 컨덕턴스 G_off [S]"; Vf "다이오드 순방향 전압 Vf [V]"; Rd "다이오드 도통 저항 R_d [Ohm]"; Goffd "다이오드 차단 컨덕턴스 [S]"
      mask help: 전력 반도체 스위치 셀 BRK. 게이트 태그 gBrk.
      settings: AttributesFormatString=gate: gBrk
      mask Display:
      | plot([0.05 0.35 ],[0.50 0.50 ],[0.35 0.65 ],[0.50 0.74 ],[0.65 0.95 ],[0.50 0.50 ]);
      | plot([0.20 0.20 0.42 ],[0.50 0.20 0.20 ],[0.58 0.80 0.80 ],[0.20 0.20 0.50 ]);
      | plot([0.42 0.58 0.58 0.42 ],[0.20 0.10 0.30 0.20 ],[0.42 0.42 ],[0.10 0.30 ]);
      | text(0.5,0.80,'BRK','horizontalAlignment','center','texmode','off');
      | port_label('LConn',1,'D');
      | port_label('RConn',1,'S');
  V_link : fl_lib/Electrical/Electrical Sensors/Voltage Sensor
  V_s : fl_lib/Electrical/Electrical Sensors/Voltage Sensor
  Xfmr_4p6to1 : fl_lib/Electrical/Electrical Elements/Ideal Transformer  n=TB.B.n  i1_specify=off  i1_priority=None  i1=0 A  i1_nominal_specify=off  i1_nominal_value=1  i1_nominal_unit=A  v1_specify=off  v1_priority=None  v1=0 V  v1_nominal_specify=off  v1_nominal_value=1  v1_nominal_unit=V  i2_specify=off  i2_priority=None  i2=0 A  i2_nominal_specify=off  i2_nominal_value=1  i2_nominal_unit=A  v2_specify=off  v2_priority=None  v2=0 V  v2_nominal_specify=off  v2_nominal_value=1  v2_nominal_unit=V
  iL_PS2SL : nesl_utility/PS-Simulink Converter  PhysicalDomain=network_engine_domain  SubClassName=ps_output  LeftPortType=input  RightPortType=output  PseudoPeriodic=off  Frequencies=[]  VectorFormat=inherit  Unit=inherit  AffineConversion=off
  ibrk_PS2SL : nesl_utility/PS-Simulink Converter  PhysicalDomain=network_engine_domain  SubClassName=ps_output  LeftPortType=input  RightPortType=output  PseudoPeriodic=off  Frequencies=[]  VectorFormat=inherit  Unit=inherit  AffineConversion=off
  ih_PS2SL : nesl_utility/PS-Simulink Converter  PhysicalDomain=network_engine_domain  SubClassName=ps_output  LeftPortType=input  RightPortType=output  PseudoPeriodic=off  Frequencies=[]  VectorFormat=inherit  Unit=inherit  AffineConversion=off
  ilink_PS2SL : nesl_utility/PS-Simulink Converter  PhysicalDomain=network_engine_domain  SubClassName=ps_output  LeftPortType=input  RightPortType=output  PseudoPeriodic=off  Frequencies=[]  VectorFormat=inherit  Unit=inherit  AffineConversion=off
  vlink_PS2SL : nesl_utility/PS-Simulink Converter  PhysicalDomain=network_engine_domain  SubClassName=ps_output  LeftPortType=input  RightPortType=output  PseudoPeriodic=off  Frequencies=[]  VectorFormat=inherit  Unit=inherit  AffineConversion=off
  vs_PS2SL : nesl_utility/PS-Simulink Converter  PhysicalDomain=network_engine_domain  SubClassName=ps_output  LeftPortType=input  RightPortType=output  PseudoPeriodic=off  Frequencies=[]  VectorFormat=inherit  Unit=inherit  AffineConversion=off
  SER : PMIOPort  Side=Left
  BUS : PMIOPort  Port=2  Side=Right
  GND : PMIOPort  Port=3  Side=Right
  tag scope: iL=global, ibrk=global, ih=global, ilink=global, vlink=global, vs=global
  wires:
  ibrk_PS2SL/1 -> [ibrk]
  vs_PS2SL/1 -> [vs]
  ih_PS2SL/1 -> [ih]
  vlink_PS2SL/1 -> [vlink]
  ilink_PS2SL/1 -> [ilink]
  iL_PS2SL/1 -> [iL]
  connections:
  C_s/RConn1 -- V_s/RConn2 -- SER/RConn1 -- HBridge/RConn2
  C_s/LConn1 -- V_s/LConn1 -- L_h/RConn1 -- BUS/RConn1 -- DAB_Primary/LConn1
  HBridge/RConn1 -- I_h/LConn1
  I_h/RConn2 -- L_h/LConn1
  HBridge/LConn1 -- C_link/LConn1 -- V_link/LConn1 -- I_link/RConn2 -- I_brk/LConn1
  HBridge/LConn2 -- C_link/RConn1 -- V_link/RConn2 -- DAB_Secondary/LConn2 -- S_BRK/RConn1
  DAB_Secondary/LConn1 -- I_link/LConn1
  DAB_Secondary/RConn1 -- Xfmr_4p6to1/RConn1
  DAB_Secondary/RConn2 -- Xfmr_4p6to1/RConn2
  DAB_Primary/RConn1 -- L_dab/LConn1
  L_dab/RConn1 -- I_Ldab/LConn1
  I_Ldab/RConn2 -- Xfmr_4p6to1/LConn1
  Xfmr_4p6to1/LConn2 -- DAB_Primary/RConn2
  DAB_Primary/LConn2 -- GND/RConn1
  I_brk/RConn2 -- R_brk/LConn1
  R_brk/RConn1 -- S_BRK/LConn1
  I_brk/RConn1 -- ibrk_PS2SL/LConn1
  V_s/RConn1 -- vs_PS2SL/LConn1
  I_h/RConn1 -- ih_PS2SL/LConn1
  V_link/RConn1 -- vlink_PS2SL/LConn1
  I_link/RConn1 -- ilink_PS2SL/LConn1
  I_Ldab/RConn1 -- iL_PS2SL/LConn1

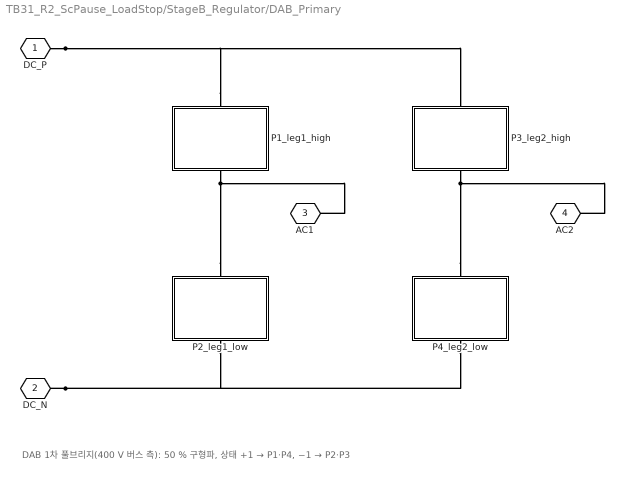
== system TB31_R2_ScPause_LoadStop/StageB_Regulator/DAB_Primary ==
  note: DAB 1차 풀브리지(400 V 버스 측): 50 % 구형파, 상태 +1 → P1·P4, −1 → P2·P3
  P1_leg1_high : Subsystem  mask(PRISM-Hub switch cell){Ron=TB.B.Ron, Goff=TB.B.Goff, Vf=TB.B.Vf, Rd=TB.B.Rd, Goffd=TB.B.Goffd, Coss=TB.B.Coss_dp}
      mask prompts: Ron "도통 저항 R_on [Ohm]"; Goff "차단 컨덕턴스 G_off [S]"; Vf "다이오드 순방향 전압 Vf [V]"; Rd "다이오드 도통 저항 R_d [Ohm]"; Goffd "다이오드 차단 컨덕턴스 [S]"; Coss "출력용량 C_oss [F]"
      mask help: 전력 반도체 스위치 셀 P1_leg1_high. 게이트 태그 gD_P1.
      settings: AttributesFormatString=gate: gD_P1
      mask Display:
      | plot([0.50 0.50 ],[0.95 0.65 ],[0.50 0.74 ],[0.65 0.35 ],[0.50 0.50 ],[0.35 0.05 ]);
      | plot([0.50 0.20 0.20 ],[0.80 0.80 0.58 ],[0.20 0.20 0.50 ],[0.42 0.20 0.20 ]);
      | plot([0.20 0.10 0.30 0.20 ],[0.58 0.42 0.42 0.58 ],[0.10 0.30 ],[0.58 0.58 ]);
      | port_label('LConn',1,'D');
      | port_label('RConn',1,'S');
  P2_leg1_low : Subsystem  mask(PRISM-Hub switch cell){Ron=TB.B.Ron, Goff=TB.B.Goff, Vf=TB.B.Vf, Rd=TB.B.Rd, Goffd=TB.B.Goffd, Coss=TB.B.Coss_dp}
      mask prompts: Ron "도통 저항 R_on [Ohm]"; Goff "차단 컨덕턴스 G_off [S]"; Vf "다이오드 순방향 전압 Vf [V]"; Rd "다이오드 도통 저항 R_d [Ohm]"; Goffd "다이오드 차단 컨덕턴스 [S]"; Coss "출력용량 C_oss [F]"
      mask help: 전력 반도체 스위치 셀 P2_leg1_low. 게이트 태그 gD_P2.
      settings: AttributesFormatString=gate: gD_P2
      mask Display:
      | plot([0.50 0.50 ],[0.95 0.65 ],[0.50 0.74 ],[0.65 0.35 ],[0.50 0.50 ],[0.35 0.05 ]);
      | plot([0.50 0.20 0.20 ],[0.80 0.80 0.58 ],[0.20 0.20 0.50 ],[0.42 0.20 0.20 ]);
      | plot([0.20 0.10 0.30 0.20 ],[0.58 0.42 0.42 0.58 ],[0.10 0.30 ],[0.58 0.58 ]);
      | port_label('LConn',1,'D');
      | port_label('RConn',1,'S');
  P3_leg2_high : Subsystem  mask(PRISM-Hub switch cell){Ron=TB.B.Ron, Goff=TB.B.Goff, Vf=TB.B.Vf, Rd=TB.B.Rd, Goffd=TB.B.Goffd, Coss=TB.B.Coss_dp}
      mask prompts: Ron "도통 저항 R_on [Ohm]"; Goff "차단 컨덕턴스 G_off [S]"; Vf "다이오드 순방향 전압 Vf [V]"; Rd "다이오드 도통 저항 R_d [Ohm]"; Goffd "다이오드 차단 컨덕턴스 [S]"; Coss "출력용량 C_oss [F]"
      mask help: 전력 반도체 스위치 셀 P3_leg2_high. 게이트 태그 gD_P3.
      settings: AttributesFormatString=gate: gD_P3
      mask Display:
      | plot([0.50 0.50 ],[0.95 0.65 ],[0.50 0.74 ],[0.65 0.35 ],[0.50 0.50 ],[0.35 0.05 ]);
      | plot([0.50 0.20 0.20 ],[0.80 0.80 0.58 ],[0.20 0.20 0.50 ],[0.42 0.20 0.20 ]);
      | plot([0.20 0.10 0.30 0.20 ],[0.58 0.42 0.42 0.58 ],[0.10 0.30 ],[0.58 0.58 ]);
      | port_label('LConn',1,'D');
      | port_label('RConn',1,'S');
  P4_leg2_low : Subsystem  mask(PRISM-Hub switch cell){Ron=TB.B.Ron, Goff=TB.B.Goff, Vf=TB.B.Vf, Rd=TB.B.Rd, Goffd=TB.B.Goffd, Coss=TB.B.Coss_dp}
      mask prompts: Ron "도통 저항 R_on [Ohm]"; Goff "차단 컨덕턴스 G_off [S]"; Vf "다이오드 순방향 전압 Vf [V]"; Rd "다이오드 도통 저항 R_d [Ohm]"; Goffd "다이오드 차단 컨덕턴스 [S]"; Coss "출력용량 C_oss [F]"
      mask help: 전력 반도체 스위치 셀 P4_leg2_low. 게이트 태그 gD_P4.
      settings: AttributesFormatString=gate: gD_P4
      mask Display:
      | plot([0.50 0.50 ],[0.95 0.65 ],[0.50 0.74 ],[0.65 0.35 ],[0.50 0.50 ],[0.35 0.05 ]);
      | plot([0.50 0.20 0.20 ],[0.80 0.80 0.58 ],[0.20 0.20 0.50 ],[0.42 0.20 0.20 ]);
      | plot([0.20 0.10 0.30 0.20 ],[0.58 0.42 0.42 0.58 ],[0.10 0.30 ],[0.58 0.58 ]);
      | port_label('LConn',1,'D');
      | port_label('RConn',1,'S');
  DC_P : PMIOPort  Side=Left
  DC_N : PMIOPort  Port=2  Side=Left
  AC1 : PMIOPort  Port=3  Side=Right
  AC2 : PMIOPort  Port=4  Side=Right
  connections:
  P1_leg1_high/LConn1 -- DC_P/RConn1 -- P3_leg2_high/LConn1
  P2_leg1_low/LConn1 -- P1_leg1_high/RConn1 -- AC1/RConn1
  P4_leg2_low/LConn1 -- P3_leg2_high/RConn1 -- AC2/RConn1
  DC_N/RConn1 -- P2_leg1_low/RConn1 -- P4_leg2_low/RConn1

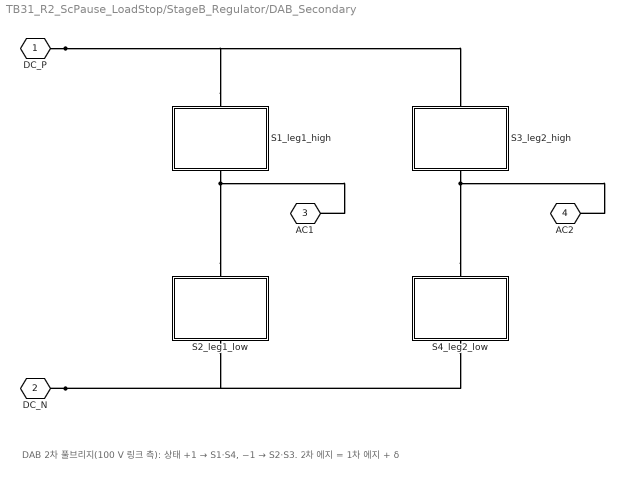
== system TB31_R2_ScPause_LoadStop/StageB_Regulator/DAB_Secondary ==
  note: DAB 2차 풀브리지(100 V 링크 측): 상태 +1 → S1·S4, −1 → S2·S3. 2차 에지 = 1차 에지 + δ
  S1_leg1_high : Subsystem  mask(PRISM-Hub switch cell){Ron=TB.B.Ron, Goff=TB.B.Goff, Vf=TB.B.Vf, Rd=TB.B.Rd, Goffd=TB.B.Goffd, Coss=TB.B.Coss_ds}
      mask prompts: Ron "도통 저항 R_on [Ohm]"; Goff "차단 컨덕턴스 G_off [S]"; Vf "다이오드 순방향 전압 Vf [V]"; Rd "다이오드 도통 저항 R_d [Ohm]"; Goffd "다이오드 차단 컨덕턴스 [S]"; Coss "출력용량 C_oss [F]"
      mask help: 전력 반도체 스위치 셀 S1_leg1_high. 게이트 태그 gD_S1.
      settings: AttributesFormatString=gate: gD_S1
      mask Display:
      | plot([0.50 0.50 ],[0.95 0.65 ],[0.50 0.74 ],[0.65 0.35 ],[0.50 0.50 ],[0.35 0.05 ]);
      | plot([0.50 0.20 0.20 ],[0.80 0.80 0.58 ],[0.20 0.20 0.50 ],[0.42 0.20 0.20 ]);
      | plot([0.20 0.10 0.30 0.20 ],[0.58 0.42 0.42 0.58 ],[0.10 0.30 ],[0.58 0.58 ]);
      | port_label('LConn',1,'D');
      | port_label('RConn',1,'S');
  S2_leg1_low : Subsystem  mask(PRISM-Hub switch cell){Ron=TB.B.Ron, Goff=TB.B.Goff, Vf=TB.B.Vf, Rd=TB.B.Rd, Goffd=TB.B.Goffd, Coss=TB.B.Coss_ds}
      mask prompts: Ron "도통 저항 R_on [Ohm]"; Goff "차단 컨덕턴스 G_off [S]"; Vf "다이오드 순방향 전압 Vf [V]"; Rd "다이오드 도통 저항 R_d [Ohm]"; Goffd "다이오드 차단 컨덕턴스 [S]"; Coss "출력용량 C_oss [F]"
      mask help: 전력 반도체 스위치 셀 S2_leg1_low. 게이트 태그 gD_S2.
      settings: AttributesFormatString=gate: gD_S2
      mask Display:
      | plot([0.50 0.50 ],[0.95 0.65 ],[0.50 0.74 ],[0.65 0.35 ],[0.50 0.50 ],[0.35 0.05 ]);
      | plot([0.50 0.20 0.20 ],[0.80 0.80 0.58 ],[0.20 0.20 0.50 ],[0.42 0.20 0.20 ]);
      | plot([0.20 0.10 0.30 0.20 ],[0.58 0.42 0.42 0.58 ],[0.10 0.30 ],[0.58 0.58 ]);
      | port_label('LConn',1,'D');
      | port_label('RConn',1,'S');
  S3_leg2_high : Subsystem  mask(PRISM-Hub switch cell){Ron=TB.B.Ron, Goff=TB.B.Goff, Vf=TB.B.Vf, Rd=TB.B.Rd, Goffd=TB.B.Goffd, Coss=TB.B.Coss_ds}
      mask prompts: Ron "도통 저항 R_on [Ohm]"; Goff "차단 컨덕턴스 G_off [S]"; Vf "다이오드 순방향 전압 Vf [V]"; Rd "다이오드 도통 저항 R_d [Ohm]"; Goffd "다이오드 차단 컨덕턴스 [S]"; Coss "출력용량 C_oss [F]"
      mask help: 전력 반도체 스위치 셀 S3_leg2_high. 게이트 태그 gD_S3.
      settings: AttributesFormatString=gate: gD_S3
      mask Display:
      | plot([0.50 0.50 ],[0.95 0.65 ],[0.50 0.74 ],[0.65 0.35 ],[0.50 0.50 ],[0.35 0.05 ]);
      | plot([0.50 0.20 0.20 ],[0.80 0.80 0.58 ],[0.20 0.20 0.50 ],[0.42 0.20 0.20 ]);
      | plot([0.20 0.10 0.30 0.20 ],[0.58 0.42 0.42 0.58 ],[0.10 0.30 ],[0.58 0.58 ]);
      | port_label('LConn',1,'D');
      | port_label('RConn',1,'S');
  S4_leg2_low : Subsystem  mask(PRISM-Hub switch cell){Ron=TB.B.Ron, Goff=TB.B.Goff, Vf=TB.B.Vf, Rd=TB.B.Rd, Goffd=TB.B.Goffd, Coss=TB.B.Coss_ds}
      mask prompts: Ron "도통 저항 R_on [Ohm]"; Goff "차단 컨덕턴스 G_off [S]"; Vf "다이오드 순방향 전압 Vf [V]"; Rd "다이오드 도통 저항 R_d [Ohm]"; Goffd "다이오드 차단 컨덕턴스 [S]"; Coss "출력용량 C_oss [F]"
      mask help: 전력 반도체 스위치 셀 S4_leg2_low. 게이트 태그 gD_S4.
      settings: AttributesFormatString=gate: gD_S4
      mask Display:
      | plot([0.50 0.50 ],[0.95 0.65 ],[0.50 0.74 ],[0.65 0.35 ],[0.50 0.50 ],[0.35 0.05 ]);
      | plot([0.50 0.20 0.20 ],[0.80 0.80 0.58 ],[0.20 0.20 0.50 ],[0.42 0.20 0.20 ]);
      | plot([0.20 0.10 0.30 0.20 ],[0.58 0.42 0.42 0.58 ],[0.10 0.30 ],[0.58 0.58 ]);
      | port_label('LConn',1,'D');
      | port_label('RConn',1,'S');
  DC_P : PMIOPort  Side=Left
  DC_N : PMIOPort  Port=2  Side=Left
  AC1 : PMIOPort  Port=3  Side=Right
  AC2 : PMIOPort  Port=4  Side=Right
  connections:
  S1_leg1_high/LConn1 -- DC_P/RConn1 -- S3_leg2_high/LConn1
  S2_leg1_low/LConn1 -- S1_leg1_high/RConn1 -- AC1/RConn1
  S4_leg2_low/LConn1 -- S3_leg2_high/RConn1 -- AC2/RConn1
  DC_N/RConn1 -- S2_leg1_low/RConn1 -- S4_leg2_low/RConn1

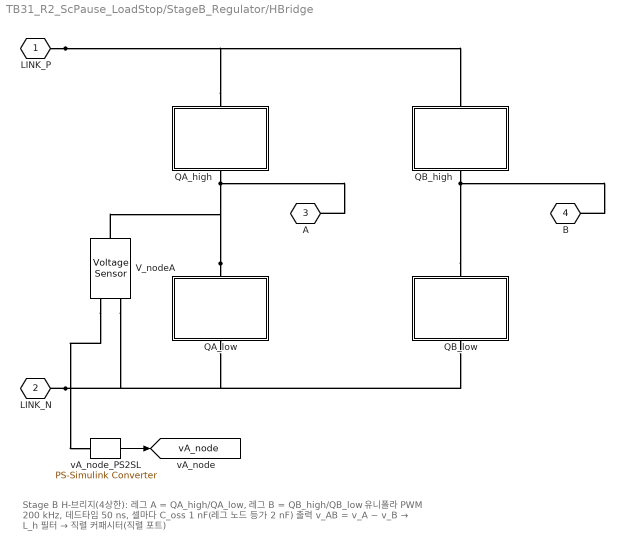
== system TB31_R2_ScPause_LoadStop/StageB_Regulator/HBridge ==
  note: Stage B H-브리지(4상한): 레그 A = QA_high/QA_low, 레그 B = QB_high/QB_low
      | 유니폴라 PWM 200 kHz, 데드타임 50 ns, 셀마다 C_oss 1 nF(레그 노드 등가 2 nF)
      | 출력 v_AB = v_A − v_B → L_h 필터 → 직렬 커패시터(직렬 포트)
  QA_high : Subsystem  mask(PRISM-Hub switch cell){Ron=TB.B.Ron, Goff=TB.B.Goff, Vf=TB.B.Vf, Rd=TB.B.Rd, Goffd=TB.B.Goffd, Coss=TB.B.Coss_h}
      mask prompts: Ron "도통 저항 R_on [Ohm]"; Goff "차단 컨덕턴스 G_off [S]"; Vf "다이오드 순방향 전압 Vf [V]"; Rd "다이오드 도통 저항 R_d [Ohm]"; Goffd "다이오드 차단 컨덕턴스 [S]"; Coss "출력용량 C_oss [F]"
      mask help: 전력 반도체 스위치 셀 QA_H. 게이트 태그 gB_AH.
      settings: AttributesFormatString=gate: gB_AH
      mask Display:
      | plot([0.50 0.50 ],[0.95 0.65 ],[0.50 0.74 ],[0.65 0.35 ],[0.50 0.50 ],[0.35 0.05 ]);
      | plot([0.50 0.20 0.20 ],[0.80 0.80 0.58 ],[0.20 0.20 0.50 ],[0.42 0.20 0.20 ]);
      | plot([0.20 0.10 0.30 0.20 ],[0.58 0.42 0.42 0.58 ],[0.10 0.30 ],[0.58 0.58 ]);
      | port_label('LConn',1,'D');
      | port_label('RConn',1,'S');
  QA_low : Subsystem  mask(PRISM-Hub switch cell){Ron=TB.B.Ron, Goff=TB.B.Goff, Vf=TB.B.Vf, Rd=TB.B.Rd, Goffd=TB.B.Goffd, Coss=TB.B.Coss_h}
      mask prompts: Ron "도통 저항 R_on [Ohm]"; Goff "차단 컨덕턴스 G_off [S]"; Vf "다이오드 순방향 전압 Vf [V]"; Rd "다이오드 도통 저항 R_d [Ohm]"; Goffd "다이오드 차단 컨덕턴스 [S]"; Coss "출력용량 C_oss [F]"
      mask help: 전력 반도체 스위치 셀 QA_L. 게이트 태그 gB_AL.
      settings: AttributesFormatString=gate: gB_AL
      mask Display:
      | plot([0.50 0.50 ],[0.95 0.65 ],[0.50 0.74 ],[0.65 0.35 ],[0.50 0.50 ],[0.35 0.05 ]);
      | plot([0.50 0.20 0.20 ],[0.80 0.80 0.58 ],[0.20 0.20 0.50 ],[0.42 0.20 0.20 ]);
      | plot([0.20 0.10 0.30 0.20 ],[0.58 0.42 0.42 0.58 ],[0.10 0.30 ],[0.58 0.58 ]);
      | port_label('LConn',1,'D');
      | port_label('RConn',1,'S');
  QB_high : Subsystem  mask(PRISM-Hub switch cell){Ron=TB.B.Ron, Goff=TB.B.Goff, Vf=TB.B.Vf, Rd=TB.B.Rd, Goffd=TB.B.Goffd, Coss=TB.B.Coss_h}
      mask prompts: Ron "도통 저항 R_on [Ohm]"; Goff "차단 컨덕턴스 G_off [S]"; Vf "다이오드 순방향 전압 Vf [V]"; Rd "다이오드 도통 저항 R_d [Ohm]"; Goffd "다이오드 차단 컨덕턴스 [S]"; Coss "출력용량 C_oss [F]"
      mask help: 전력 반도체 스위치 셀 QB_H. 게이트 태그 gB_BH.
      settings: AttributesFormatString=gate: gB_BH
      mask Display:
      | plot([0.50 0.50 ],[0.95 0.65 ],[0.50 0.74 ],[0.65 0.35 ],[0.50 0.50 ],[0.35 0.05 ]);
      | plot([0.50 0.20 0.20 ],[0.80 0.80 0.58 ],[0.20 0.20 0.50 ],[0.42 0.20 0.20 ]);
      | plot([0.20 0.10 0.30 0.20 ],[0.58 0.42 0.42 0.58 ],[0.10 0.30 ],[0.58 0.58 ]);
      | port_label('LConn',1,'D');
      | port_label('RConn',1,'S');
  QB_low : Subsystem  mask(PRISM-Hub switch cell){Ron=TB.B.Ron, Goff=TB.B.Goff, Vf=TB.B.Vf, Rd=TB.B.Rd, Goffd=TB.B.Goffd, Coss=TB.B.Coss_h}
      mask prompts: Ron "도통 저항 R_on [Ohm]"; Goff "차단 컨덕턴스 G_off [S]"; Vf "다이오드 순방향 전압 Vf [V]"; Rd "다이오드 도통 저항 R_d [Ohm]"; Goffd "다이오드 차단 컨덕턴스 [S]"; Coss "출력용량 C_oss [F]"
      mask help: 전력 반도체 스위치 셀 QB_L. 게이트 태그 gB_BL.
      settings: AttributesFormatString=gate: gB_BL
      mask Display:
      | plot([0.50 0.50 ],[0.95 0.65 ],[0.50 0.74 ],[0.65 0.35 ],[0.50 0.50 ],[0.35 0.05 ]);
      | plot([0.50 0.20 0.20 ],[0.80 0.80 0.58 ],[0.20 0.20 0.50 ],[0.42 0.20 0.20 ]);
      | plot([0.20 0.10 0.30 0.20 ],[0.58 0.42 0.42 0.58 ],[0.10 0.30 ],[0.58 0.58 ]);
      | port_label('LConn',1,'D');
      | port_label('RConn',1,'S');
  V_nodeA : fl_lib/Electrical/Electrical Sensors/Voltage Sensor
  vA_node_PS2SL : nesl_utility/PS-Simulink Converter  PhysicalDomain=network_engine_domain  SubClassName=ps_output  LeftPortType=input  RightPortType=output  PseudoPeriodic=off  Frequencies=[]  VectorFormat=inherit  Unit=inherit  AffineConversion=off
  LINK_P : PMIOPort  Side=Left
  LINK_N : PMIOPort  Port=2  Side=Left
  A : PMIOPort  Port=3  Side=Right
  B : PMIOPort  Port=4  Side=Right
  tag scope: vA_node=global
  wires:
  vA_node_PS2SL/1 -> [vA_node]
  connections:
  QA_high/LConn1 -- LINK_P/RConn1 -- QB_high/LConn1
  QA_high/RConn1 -- A/RConn1 -- QA_low/LConn1 -- V_nodeA/LConn1
  QB_low/LConn1 -- QB_high/RConn1 -- B/RConn1
  QA_low/RConn1 -- QB_low/RConn1 -- LINK_N/RConn1 -- V_nodeA/RConn2
  V_nodeA/RConn1 -- vA_node_PS2SL/LConn1

== system TB31_R2_ScPause_LoadStop/StageB_Regulator/S_BRK ==
  note: 스위치 셀: 이상 스위치(R_on, G_off) + 역병렬 바디 다이오드(Vf, R_d)
      | 게이트: 전역 태그 "gBrk" (> 0.5 이면 도통)
  D_body : fl_lib/Electrical/Electrical Elements/Diode  Vf=Vf V  Ron=Rd Ohm  Goff=Goffd 1/Ohm  i_specify=off  i_priority=None  i=0 A  i_nominal_specify=off  i_nominal_value=1  i_nominal_unit=A  v_specify=off  v_priority=None  v=0 V  v_nominal_specify=off  v_nominal_value=1  v_nominal_unit=V
  Gate_PS : nesl_utility/Simulink-PS Converter  PhysicalDomain=network_engine_domain  SubClassName=ps_input  LeftPortType=input  RightPortType=output  PseudoPeriodic=off  Frequencies=[]  NoiseDistribution=none  NoiseParameters=[]  Unit=1  AffineConversion=off  FilteringAndDerivatives=zero  SimscapeFilterOrder=1  InputFilterTimeConstant=0.001  UdotUserProvided=0
  SW : fl_lib/Electrical/Electrical Elements/Switch  R_closed=Ron Ohm  G_open=Goff 1/Ohm  Threshold=0.5  i_specify=off  i_priority=None  i=0 A  i_nominal_specify=off  i_nominal_value=1  i_nominal_unit=A  v_specify=off  v_priority=None  v=0 V  v_nominal_specify=off  v_nominal_value=1  v_nominal_unit=V
  D : PMIOPort  Side=Left
  S : PMIOPort  Port=2  Side=Right
  wires:
  [gBrk] -> Gate_PS/1
  connections:
  Gate_PS/RConn1 -- SW/RConn1
  SW/LConn1 -- D/RConn1 -- D_body/RConn1
  S/RConn1 -- SW/RConn2 -- D_body/LConn1

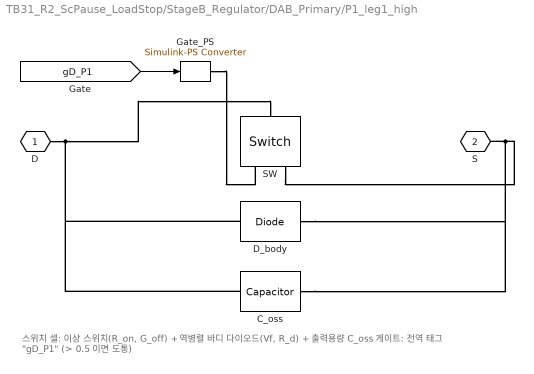
== system TB31_R2_ScPause_LoadStop/StageB_Regulator/DAB_Primary/P1_leg1_high ==
  note: 스위치 셀: 이상 스위치(R_on, G_off) + 역병렬 바디 다이오드(Vf, R_d) + 출력용량 C_oss
      | 게이트: 전역 태그 "gD_P1" (> 0.5 이면 도통)
  C_oss : fl_lib/Electrical/Electrical Elements/Capacitor  c=Coss F  r=1e-6 Ohm  g=0 1/Ohm  i_specify=off  i_priority=None  i=0 A  i_nominal_specify=off  i_nominal_value=1  i_nominal_unit=A  v_specify=off  v_priority=None  v=0 V  v_nominal_specify=off  v_nominal_value=1  v_nominal_unit=V  vc_specify=off  vc_priority=High  vc=0 V  vc_nominal_specify=off  vc_nominal_value=1  vc_nominal_unit=V
  D_body : fl_lib/Electrical/Electrical Elements/Diode  Vf=Vf V  Ron=Rd Ohm  Goff=Goffd 1/Ohm  i_specify=off  i_priority=None  i=0 A  i_nominal_specify=off  i_nominal_value=1  i_nominal_unit=A  v_specify=off  v_priority=None  v=0 V  v_nominal_specify=off  v_nominal_value=1  v_nominal_unit=V
  Gate_PS : nesl_utility/Simulink-PS Converter  PhysicalDomain=network_engine_domain  SubClassName=ps_input  LeftPortType=input  RightPortType=output  PseudoPeriodic=off  Frequencies=[]  NoiseDistribution=none  NoiseParameters=[]  Unit=1  AffineConversion=off  FilteringAndDerivatives=zero  SimscapeFilterOrder=1  InputFilterTimeConstant=0.001  UdotUserProvided=0
  SW : fl_lib/Electrical/Electrical Elements/Switch  R_closed=Ron Ohm  G_open=Goff 1/Ohm  Threshold=0.5  i_specify=off  i_priority=None  i=0 A  i_nominal_specify=off  i_nominal_value=1  i_nominal_unit=A  v_specify=off  v_priority=None  v=0 V  v_nominal_specify=off  v_nominal_value=1  v_nominal_unit=V
  D : PMIOPort  Side=Left
  S : PMIOPort  Port=2  Side=Right
  wires:
  [gD_P1] -> Gate_PS/1
  connections:
  Gate_PS/RConn1 -- SW/RConn1
  SW/LConn1 -- D/RConn1 -- D_body/RConn1 -- C_oss/LConn1
  SW/RConn2 -- D_body/LConn1 -- S/RConn1 -- C_oss/RConn1

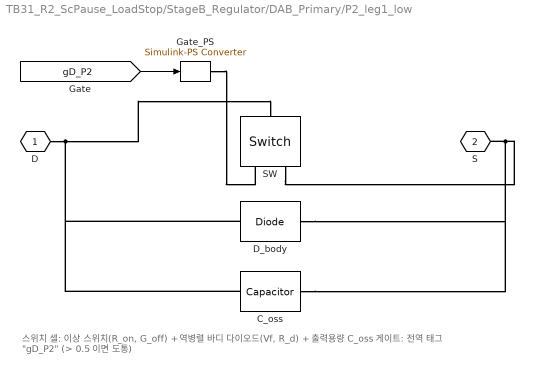
== system TB31_R2_ScPause_LoadStop/StageB_Regulator/DAB_Primary/P2_leg1_low ==
  note: 스위치 셀: 이상 스위치(R_on, G_off) + 역병렬 바디 다이오드(Vf, R_d) + 출력용량 C_oss
      | 게이트: 전역 태그 "gD_P2" (> 0.5 이면 도통)
  C_oss : fl_lib/Electrical/Electrical Elements/Capacitor  c=Coss F  r=1e-6 Ohm  g=0 1/Ohm  i_specify=off  i_priority=None  i=0 A  i_nominal_specify=off  i_nominal_value=1  i_nominal_unit=A  v_specify=off  v_priority=None  v=0 V  v_nominal_specify=off  v_nominal_value=1  v_nominal_unit=V  vc_specify=off  vc_priority=High  vc=0 V  vc_nominal_specify=off  vc_nominal_value=1  vc_nominal_unit=V
  D_body : fl_lib/Electrical/Electrical Elements/Diode  Vf=Vf V  Ron=Rd Ohm  Goff=Goffd 1/Ohm  i_specify=off  i_priority=None  i=0 A  i_nominal_specify=off  i_nominal_value=1  i_nominal_unit=A  v_specify=off  v_priority=None  v=0 V  v_nominal_specify=off  v_nominal_value=1  v_nominal_unit=V
  Gate_PS : nesl_utility/Simulink-PS Converter  PhysicalDomain=network_engine_domain  SubClassName=ps_input  LeftPortType=input  RightPortType=output  PseudoPeriodic=off  Frequencies=[]  NoiseDistribution=none  NoiseParameters=[]  Unit=1  AffineConversion=off  FilteringAndDerivatives=zero  SimscapeFilterOrder=1  InputFilterTimeConstant=0.001  UdotUserProvided=0
  SW : fl_lib/Electrical/Electrical Elements/Switch  R_closed=Ron Ohm  G_open=Goff 1/Ohm  Threshold=0.5  i_specify=off  i_priority=None  i=0 A  i_nominal_specify=off  i_nominal_value=1  i_nominal_unit=A  v_specify=off  v_priority=None  v=0 V  v_nominal_specify=off  v_nominal_value=1  v_nominal_unit=V
  D : PMIOPort  Side=Left
  S : PMIOPort  Port=2  Side=Right
  wires:
  [gD_P2] -> Gate_PS/1
  connections:
  Gate_PS/RConn1 -- SW/RConn1
  SW/LConn1 -- D/RConn1 -- D_body/RConn1 -- C_oss/LConn1
  SW/RConn2 -- D_body/LConn1 -- S/RConn1 -- C_oss/RConn1
